simulink library "lib_AC_GFM"  (R2026a)
settings: Solver=VariableStepAuto
undefined symbols (not defined in the file): block_buses, block_idx, block_toM, buses_lf, fref, iC, invL, iR, iTf, op_GFM
libraries: simulink x4
(part 2 of 2)

== system lib_AC_GFM/GFM/VCC/dynamic_limiting/PIvd ==
  ref : Inport
  y : Inport  Port=2
  anti_windup : Inport  Port=3
  Gain : Gain  Gain=Bext
  Gain1 : Gain  Gain=1./Text
  Gain2 : Gain  Gain=Kext
  I : Integrator  InitialCondition=op_GFM.VCC_dynamic_limiting_PIvd_I
  Product : Product
  Scope : Scope
      settings: ActiveDisplayYMinimum=-5E-5  ActiveDisplayYMaximum=0.00079  DataLoggingVariableName=ScopeData5
  Scope1 : Scope
      settings: ActiveDisplayYMinimum=-0.29497  ActiveDisplayYMaximum=2.2504  DataLoggingVariableName=ScopeData7
  Sum : Sum  Inputs=++|
  Sum1 : Sum  Inputs=|+-
  Sum6 : Sum  Inputs=|+-
  Out1 : Outport
  wires:
  y/1 -> Sum1/2, Sum6/2
  ref/1 -> Gain/1, Sum6/1
  Gain/1 -> Sum1/1
  Sum/1 -> Gain2/1
  Sum1/1 -> Sum/1
  Sum6/1 -> Scope1/1, Gain1/1
  Product/1 -> I/1
  I/1 -> Scope/1, Sum/2
  Gain2/1 -> Out1/1
  Gain1/1 -> Product/1
  anti_windup/1 -> Product/2

== system lib_AC_GFM/GFM/VCC/dynamic_limiting/PIvq ==
  ref : Inport
  y : Inport  Port=2
  anti_windup : Inport  Port=3
  Gain : Gain  Gain=Bext
  Gain1 : Gain  Gain=1./Text
  Gain2 : Gain  Gain=Kext
  I : Integrator  InitialCondition=op_GFM.VCC_dynamic_limiting_PIvq_I
  Product : Product
  Sum : Sum  Inputs=++|
  Sum1 : Sum  Inputs=|+-
  Sum6 : Sum  Inputs=|+-
  Out1 : Outport
  wires:
  Gain2/1 -> Out1/1
  I/1 -> Sum/2
  Product/1 -> I/1
  Sum6/1 -> Gain1/1
  Sum1/1 -> Sum/1
  Sum/1 -> Gain2/1
  Gain/1 -> Sum1/1
  ref/1 -> Sum6/1, Gain/1
  y/1 -> Sum6/2, Sum1/2
  Gain1/1 -> Product/1
  anti_windup/1 -> Product/2

== system lib_AC_GFM/GFM/VCC/dynamic_limiting/RC ==
  note: 1) Add Subsystem or Model blocks as valid variant choices.
      | 2) You cannot connect blocks at this level. At simulation, connectivity is automatically
      | determined, based on the active variant and port name matching.
  i_d_in : Inport
  i_d_out : Inport  Port=2
  i_q_in : Inport  Port=3
  i_q_out : Inport  Port=4
  omega : Inport  Port=5
  dynamic : Subsystem  VariantControl=rc_mode == 1
  static : Subsystem  VariantControl=rc_mode == 2
  static omega : Subsystem  VariantControl=(default)
  vd : Outport
  vq : Outport  Port=2

== system lib_AC_GFM/GFM/VCC/dynamic_limiting/RL ==
  note: 1) Add Subsystem or Model blocks as valid variant choices.
      | 2) You cannot connect blocks at this level. At simulation, connectivity is automatically
      | determined, based on the active variant and port name matching.
  v_in_d : Inport
  v_out_d : Inport  Port=2
  v_in_q : Inport  Port=3
  v_out_q : Inport  Port=4
  omega : Inport  Port=5
  dynamic : Subsystem  VariantControl=rl_mode == 1
      settings: PortSchema="{\"entries\":[{\"content\":{\"sides\":[{\"content\":{\"connectorIds\":[\"In1\"]},\"type\":\"ConnectorPlacement.EquallySpacedRectSide\",\"uuid\":\"63966e24-f9e7-4b2d-b456-7f4ea5e3f230\"},{\"content\":{\"connectorIds\":[\"In2\",\"In3\",\"In4\",\"In5\",\"Out1\",\"Out2\"],\"side\":\"RIGHT\"},\"type\":\"ConnectorPlacement.EquallySpacedRectSide\",\"uuid\":\"ded6ef04-52fd-47df-8e49-cf16b827098d\"},{\"content\":{\"side\":\"TOP\"},\"type\":\"ConnectorPlacement.EquallySpacedRectSide\",\"uuid\":\"f940a985-fa23-4968-ad44-1d76d0e20c6a\"}]},\"type\":\"ConnectorPlacement.EquallySpacedConnector\",\"uuid\":\"20f61d3c-9af2-4982-98ea-af4910e61c9c\"}],\"packageUris\":[\"http://schema.mathworks.com/mf0/Connector/R2020b\"],\"version\":\"1.0\"}"
  static : Subsystem  VariantControl=rl_mode == 2
  static_omega : Subsystem  VariantControl=(default)
  id : Outport
  iq : Outport  Port=2

== system lib_AC_GFM/GFM/VCC/dynamic_limiting/VI ==
  id : Inport
  iq : Inport  Port=2
  Gain : Gain  Gain=L
  Gain1 : Gain  Gain=R
  Gain2 : Gain  Gain=L
  Gain3 : Gain  Gain=R
  LPF_omega : Subsystem
  LPF_omega1 : Subsystem
  Sum : Sum  Inputs=-+|
  Sum1 : Sum  Inputs=|--
  WOF_d : Subsystem  Variant=on
  WOF_q : Subsystem  Variant=on
  vd : Outport
  vq : Outport  Port=2
  wires:
  WOF_q/1(Out1) -> Gain/1, Gain3/1
  iq/1 -> WOF_q/1(In1)
  WOF_d/1(Out1) -> Gain1/1, Gain2/1
  id/1 -> WOF_d/1(In1)
  Sum1/1 -> LPF_omega1/1(in)
  Sum/1 -> LPF_omega/1(in)
  Gain3/1 -> Sum1/2
  Gain1/1 -> Sum/1
  Gain2/1 -> Sum1/1
  Gain/1 -> Sum/2
  LPF_omega/1(out) -> vd/1
  LPF_omega1/1(out) -> vq/1

== system lib_AC_GFM/GFM/VI/WOF_d/Active ==
  In1 : Inport
  Impl : Subsystem
  Out1 : Outport
  wires:
  Impl/1(Out1) -> Out1/1
  In1/1 -> Impl/1(In1)

== system lib_AC_GFM/GFM/VI/WOF_d/Bypass ==
  In1 : Inport
  Out1 : Outport
  wires:
  In1/1 -> Out1/1

== system lib_AC_GFM/GFM/VI/WOF_q/Active ==
  In1 : Inport
  Impl : Subsystem
  Out1 : Outport
  wires:
  Impl/1(Out1) -> Out1/1
  In1/1 -> Impl/1(In1)

== system lib_AC_GFM/GFM/VI/WOF_q/Bypass ==
  In1 : Inport
  Out1 : Outport
  wires:
  In1/1 -> Out1/1

== system lib_AC_GFM/GFM/PC/LPF_P/Active/Impl ==
  P : Inport
  Gain : Gain  Gain=iTf
  I : Integrator  InitialCondition=op_GFM.PC_LPF_P_Active_Impl_I
  Sum4 : Sum  Inputs=|+-
  P_f : Outport
  wires:
  I/1 -> Sum4/2, P_f/1
  P/1 -> Sum4/1
  Sum4/1 -> Gain/1
  Gain/1 -> I/1

== system lib_AC_GFM/GFM/PC/LPF_Q/Active/Impl ==
  Q : Inport
  Gain : Gain  Gain=iTf
  I : Integrator  InitialCondition=op_GFM.PC_LPF_Q_Active_Impl_I
  Sum4 : Sum  Inputs=|+-
  Q_f : Outport
  wires:
  Sum4/1 -> Gain/1
  I/1 -> Sum4/2, Q_f/1
  Q/1 -> Sum4/1
  Gain/1 -> I/1

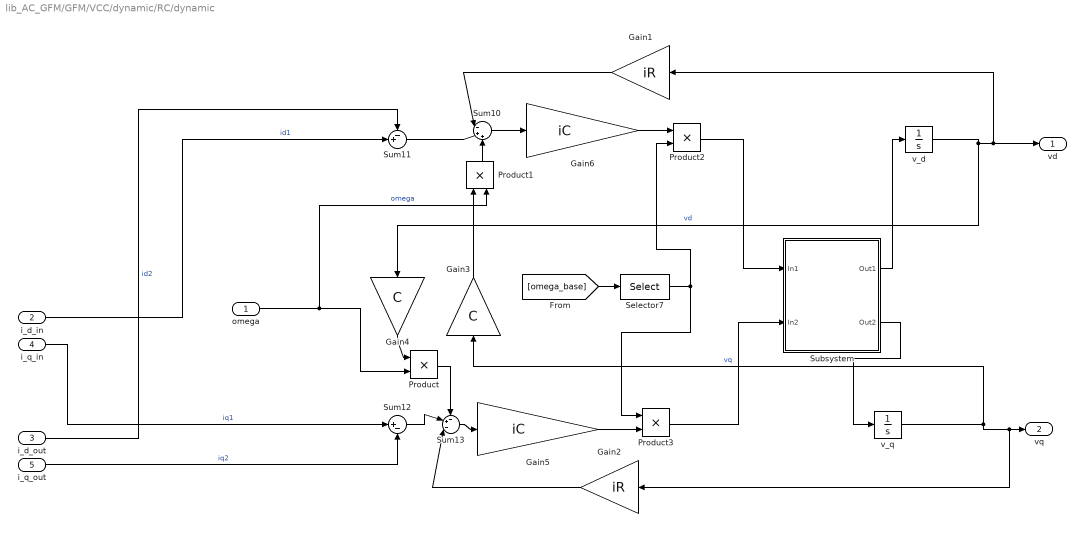
== system lib_AC_GFM/GFM/VCC/dynamic/RC/dynamic ==
  omega : Inport
  i_d_in : Inport  Port=2
  i_d_out : Inport  Port=3
  i_q_in : Inport  Port=4
  i_q_out : Inport  Port=5
  Gain1 : Gain  Gain=iR
  Gain2 : Gain  Gain=iR
  Gain3 : Gain  Gain=C
  Gain4 : Gain  Gain=C
  Gain5 : Gain  Gain=iC
  Gain6 : Gain  Gain=iC
  Product{,1..3} (4 alike) : Product
  Selector7 : Selector  InputPortWidth=length(fref.ref_units)  IndexOptions=Index vector (dialog)  Indices=block_fref  OutputSizes=1
  Subsystem : Subsystem
  Sum10 : Sum  Inputs=|-++
  Sum11 : Sum  Inputs=-+|
  Sum12 : Sum  Inputs=|+-
  Sum13 : Sum  Inputs=-+-|
  v_d : Integrator  InitialCondition=op_GFM.VCC_dynamic_RC_dynamic_v_d
  v_q : Integrator  InitialCondition=op_GFM.VCC_dynamic_RC_dynamic_v_q
  vd : Outport
  vq : Outport  Port=2
  wires:
  Sum10/1 -> Gain6/1
  Gain3/1 -> Product1/1
  v_q/1 -> vq/1, Gain2/1, Gain3/1  "vq"
  Product1/1 -> Sum10/3
  Gain4/1 -> Product/1
  Gain2/1 -> Sum13/3
  Product/1 -> Sum13/1
  Sum11/1 -> Sum10/2
  omega/1 -> Product/2, Product1/2  "omega"
  Sum13/1 -> Gain5/1
  Gain1/1 -> Sum10/1
  Sum12/1 -> Sum13/2
  v_d/1 -> Gain4/1, Gain1/1, vd/1  "vd"
  i_d_in/1 -> Sum11/2  "id1"
  i_d_out/1 -> Sum11/1  "id2"
  i_q_in/1 -> Sum12/1  "iq1"
  i_q_out/1 -> Sum12/2  "iq2"
  [omega_base] -> Selector7/1
  Gain6/1 -> Product2/1
  Product2/1 -> Subsystem/1(In1)
  Selector7/1 -> Product2/2, Product3/1
  Gain5/1 -> Product3/2
  Subsystem/1(Out1) -> v_d/1
  Product3/1 -> Subsystem/2(In2)
  Subsystem/2(Out2) -> v_q/1

== system lib_AC_GFM/GFM/VCC/dynamic/RC/static ==
  omega : Inport
  i_d_in : Inport  Port=2
  i_d_out : Inport  Port=3
  i_q_in : Inport  Port=4
  i_q_out : Inport  Port=5
  Constant : Constant  Value=iR.^2
  Constant1 : Constant
  Divide : Product  Inputs=*/
  Gain : Gain  Gain=C
  Gain1 : Gain  Gain=iR
  Gain2 : Gain  Gain=iR
  Product{,1..5} (6 alike) : Product
  Sum : Sum  Inputs=|++
  Sum1 : Sum  Inputs=|-+
  Sum2 : Sum  Inputs=|+-
  Sum3 : Sum  Inputs=|++
  Sum4 : Sum  Inputs=|-+
  vd : Outport
  vq : Outport  Port=2
  wires:
  Product5/1 -> Sum4/2
  Gain2/1 -> Product5/2
  Product4/1 -> Sum4/1
  Product2/1 -> Product3/1, Product4/2
  Product3/1 -> Sum3/2
  Product1/1 -> Sum3/1
  Divide/1 -> Product2/1, Gain1/1, Product5/1
  Gain1/1 -> Product1/2
  Sum2/1 -> Product3/2, Gain2/1  "iq"
  Sum1/1 -> Product4/1, Product1/1  "id"
  Constant1/1 -> Divide/1
  Product/1 -> Sum/2
  Gain/1 -> Product/1, Product/2, Product2/2
  Sum/1 -> Divide/2
  Constant/1 -> Sum/1
  Sum4/1 -> vq/1  "vq"
  Sum3/1 -> vd/1  "vd"
  omega/1 -> Gain/1  "omega"
  i_d_in/1 -> Sum1/2  "id1"
  i_q_in/1 -> Sum1/1  "id2"
  i_d_out/1 -> Sum2/1  "iq1"
  i_q_out/1 -> Sum2/2  "iq2"

== system lib_AC_GFM/GFM/VCC/dynamic/RC/static omega ==
  i_d_in : Inport
  i_d_out : Inport  Port=2
  i_q_in : Inport  Port=3
  i_q_out : Inport  Port=4
  Gain : Gain  Gain=1./(iR.^2+C.^2)
  Gain2 : Gain  Gain=1./(iR.^2+C.^2)
  Gain3 : Gain  Gain=iR
  Gain4 : Gain  Gain=C
  Gain5 : Gain  Gain=iR
  Gain6 : Gain  Gain=C
  Sum : Sum  Inputs=|++
  Sum1 : Sum  Inputs=|+-
  Sum2 : Sum  Inputs=|+-
  Sum4 : Sum  Inputs=|-+
  vd : Outport
  vq : Outport  Port=2
  wires:
  i_q_in/1 -> Sum2/1  "iq1"
  Sum1/1 -> Gain/1  "id"
  Sum2/1 -> Gain2/1  "iq"
  i_q_out/1 -> Sum2/2  "iq2"
  i_d_in/1 -> Sum1/1  "id"
  i_d_out/1 -> Sum1/2
  Gain/1 -> Gain4/1, Gain3/1
  Gain2/1 -> Gain6/1, Gain5/1
  Gain3/1 -> Sum/1
  Gain6/1 -> Sum/2
  Gain4/1 -> Sum4/1
  Gain5/1 -> Sum4/2
  Sum4/1 -> vq/1
  Sum/1 -> vd/1

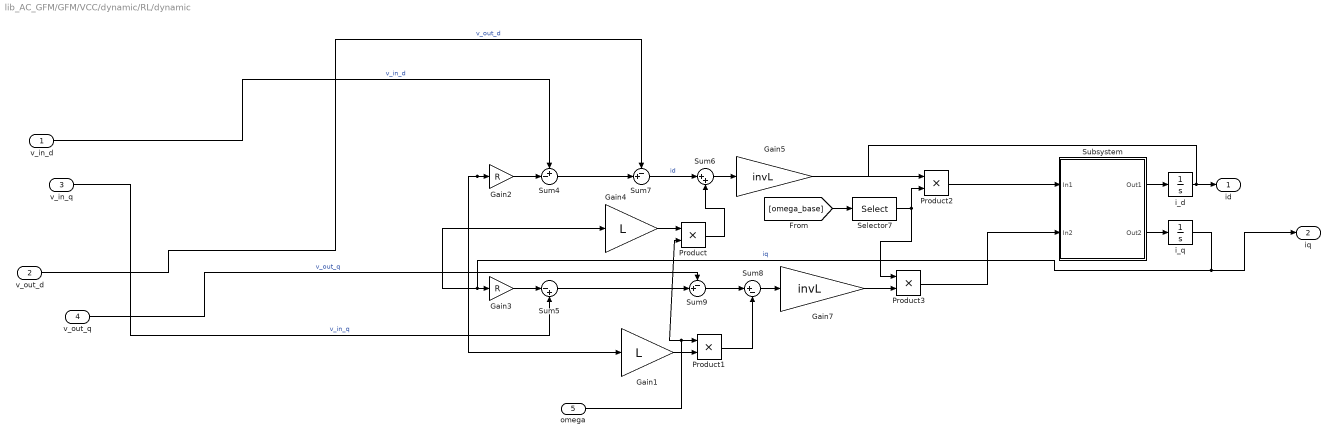
== system lib_AC_GFM/GFM/VCC/dynamic/RL/dynamic ==
  v_in_d : Inport
  v_out_d : Inport  Port=2
  v_in_q : Inport  Port=3
  v_out_q : Inport  Port=4
  omega : Inport  Port=5
  Gain1 : Gain  Gain=L
  Gain2 : Gain  Gain=R
  Gain3 : Gain  Gain=R
  Gain4 : Gain  Gain=L
  Gain5 : Gain  Gain=invL
  Gain7 : Gain  Gain=invL
  Product{,1..3} (4 alike) : Product
  Selector7 : Selector  InputPortWidth=length(fref.ref_units)  IndexOptions=Index vector (dialog)  Indices=block_fref  OutputSizes=1
  Subsystem : Subsystem
  Sum4 : Sum  Inputs=+-|
  Sum5 : Sum  Inputs=|-+
  Sum6 : Sum  Inputs=|++
  Sum7 : Sum  Inputs=-+|
  Sum8 : Sum  Inputs=|+-
  Sum9 : Sum  Inputs=-+|
  i_d : Integrator  InitialCondition=op_GFM.VCC_dynamic_RL_dynamic_i_d
  i_q : Integrator  InitialCondition=op_GFM.VCC_dynamic_RL_dynamic_i_q
  id : Outport
  iq : Outport  Port=2
  wires:
  v_out_q/1 -> Sum9/1  "v_out_q"
  v_out_d/1 -> Sum7/1  "v_out_d"
  Sum9/1 -> Sum8/1
  Gain1/1 -> Product1/2
  i_q/1 -> Gain4/1, Gain3/1, iq/1  "iq"
  Gain7/1 -> Product3/2
  Sum5/1 -> Sum9/2
  Gain3/1 -> Sum5/1
  Sum7/1 -> Sum6/1
  Gain4/1 -> Product/1
  Product1/1 -> Sum8/2
  Sum4/1 -> Sum7/2
  Sum8/1 -> Gain7/1
  Product/1 -> Sum6/2
  Sum6/1 -> Gain5/1
  i_d/1 -> id/1, Gain1/1, Gain2/1  "id"
  Gain2/1 -> Sum4/2
  v_in_d/1 -> Sum4/1  "v_in_d"
  v_in_q/1 -> Sum5/2  "v_in_q"
  omega/1 -> Product/2, Product1/1
  Gain5/1 -> Product2/1
  Product2/1 -> Subsystem/1(In1)
  Selector7/1 -> Product2/2, Product3/1
  [omega_base] -> Selector7/1
  Product3/1 -> Subsystem/2(In2)
  Subsystem/1(Out1) -> i_d/1
  Subsystem/2(Out2) -> i_q/1

== system lib_AC_GFM/GFM/VCC/dynamic/RL/static ==
  v_in_d : Inport
  v_out_d : Inport  Port=2
  v_in_q : Inport  Port=3
  v_out_q : Inport  Port=4
  omega : Inport  Port=5
  Constant : Constant  Value=R.^2
  Constant1 : Constant
  Divide : Product  Inputs=*/
  Gain : Gain  Gain=L
  Gain1 : Gain  Gain=R
  Gain2 : Gain  Gain=R
  Product{,1..5} (6 alike) : Product
  Sum : Sum  Inputs=|++
  Sum1 : Sum  Inputs=|+-
  Sum2 : Sum  Inputs=|+-
  Sum3 : Sum  Inputs=|++
  Sum4 : Sum  Inputs=|-+
  id : Outport
  iq : Outport  Port=2
  wires:
  omega/1 -> Gain/1  "omega"
  v_in_d/1 -> Sum1/1  "v_in_d"
  v_out_q/1 -> Sum2/2  "v_out_q"
  Sum4/1 -> iq/1  "iq"
  Sum3/1 -> id/1  "id"
  Gain1/1 -> Product1/2
  Product2/1 -> Product4/2, Product3/1
  Product4/1 -> Sum4/1
  Divide/1 -> Gain2/1, Gain1/1, Product2/1
  Sum1/1 -> Product1/1, Product4/1  "vd"
  Product3/1 -> Sum3/2
  Constant1/1 -> Divide/1
  Gain/1 -> Product/2, Product/1, Product2/2
  Sum2/1 -> Product5/1, Product3/2  "vq"
  Constant/1 -> Sum/1
  Product5/1 -> Sum4/2
  Product1/1 -> Sum3/1
  Product/1 -> Sum/2
  Gain2/1 -> Product5/2
  Sum/1 -> Divide/2
  v_out_d/1 -> Sum1/2  "v_out_d"
  v_in_q/1 -> Sum2/1  "v_in_q"

== system lib_AC_GFM/GFM/VCC/dynamic/RL/static_omega ==
  v_in_d : Inport
  v_out_d : Inport  Port=2
  v_in_q : Inport  Port=3
  v_out_q : Inport  Port=4
  Gain : Gain  Gain=1./(R.^2+L.^2)
  Gain2 : Gain  Gain=1./(R.^2+L.^2)
  Gain3 : Gain  Gain=R
  Gain4 : Gain  Gain=L
  Gain5 : Gain  Gain=L
  Gain6 : Gain  Gain=R
  Sum : Sum  Inputs=|++
  Sum1 : Sum  Inputs=|+-
  Sum2 : Sum  Inputs=|+-
  Sum3 : Sum  Inputs=|-+
  id : Outport
  iq : Outport  Port=2
  wires:
  v_in_q/1 -> Sum2/1  "v_in_q"
  v_in_d/1 -> Sum1/1  "v_in_d"
  v_out_q/1 -> Sum2/2  "v_out_q"
  v_out_d/1 -> Sum1/2  "v_out_d"
  Sum1/1 -> Gain/1  "vd"
  Sum2/1 -> Gain2/1  "vq"
  Gain/1 -> Gain5/1, Gain3/1
  Gain3/1 -> Sum/1
  Gain4/1 -> Sum/2
  Gain2/1 -> Gain6/1, Gain4/1
  Sum/1 -> id/1
  Gain5/1 -> Sum3/1
  Sum3/1 -> iq/1
  Gain6/1 -> Sum3/2

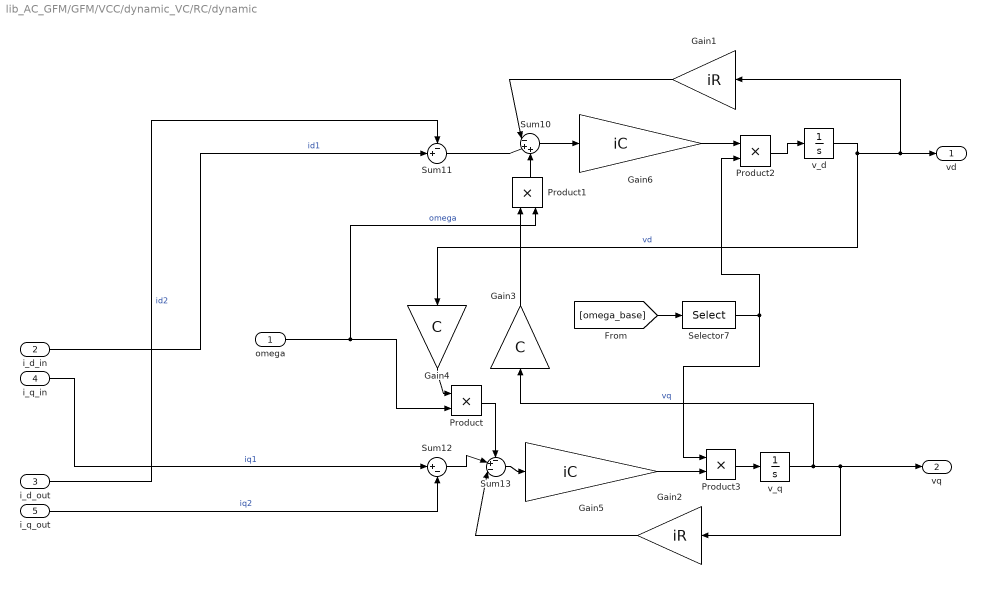
== system lib_AC_GFM/GFM/VCC/dynamic_VC/RC/dynamic ==
  omega : Inport
  i_d_in : Inport  Port=2
  i_d_out : Inport  Port=3
  i_q_in : Inport  Port=4
  i_q_out : Inport  Port=5
  Gain1 : Gain  Gain=iR
  Gain2 : Gain  Gain=iR
  Gain3 : Gain  Gain=C
  Gain4 : Gain  Gain=C
  Gain5 : Gain  Gain=iC
  Gain6 : Gain  Gain=iC
  Product{,1..3} (4 alike) : Product
  Selector7 : Selector  InputPortWidth=length(fref.ref_units)  IndexOptions=Index vector (dialog)  Indices=block_fref  OutputSizes=1
  Sum10 : Sum  Inputs=|-++
  Sum11 : Sum  Inputs=-+|
  Sum12 : Sum  Inputs=|+-
  Sum13 : Sum  Inputs=-+-|
  v_d : Integrator  InitialCondition=op_GFM.VCC_dynamic_VC_RC_dynamic_v_d
  v_q : Integrator  InitialCondition=op_GFM.VCC_dynamic_VC_RC_dynamic_v_q
  vd : Outport
  vq : Outport  Port=2
  wires:
  Sum10/1 -> Gain6/1
  Gain3/1 -> Product1/1
  v_q/1 -> vq/1, Gain2/1, Gain3/1  "vq"
  Product1/1 -> Sum10/3
  Gain4/1 -> Product/1
  Gain2/1 -> Sum13/3
  Product/1 -> Sum13/1
  Sum11/1 -> Sum10/2
  omega/1 -> Product/2, Product1/2  "omega"
  Sum13/1 -> Gain5/1
  Gain1/1 -> Sum10/1
  Sum12/1 -> Sum13/2
  v_d/1 -> Gain4/1, vd/1, Gain1/1  "vd"
  i_d_in/1 -> Sum11/2  "id1"
  i_d_out/1 -> Sum11/1  "id2"
  i_q_in/1 -> Sum12/1  "iq1"
  i_q_out/1 -> Sum12/2  "iq2"
  [omega_base] -> Selector7/1
  Gain6/1 -> Product2/1
  Product2/1 -> v_d/1
  Selector7/1 -> Product2/2, Product3/1
  Product3/1 -> v_q/1
  Gain5/1 -> Product3/2

== system lib_AC_GFM/GFM/VCC/dynamic_VC/RC/static ==
  omega : Inport
  i_d_in : Inport  Port=2
  i_d_out : Inport  Port=3
  i_q_in : Inport  Port=4
  i_q_out : Inport  Port=5
  Constant : Constant  Value=iR.^2
  Constant1 : Constant
  Divide : Product  Inputs=*/
  Gain : Gain  Gain=C
  Gain1 : Gain  Gain=iR
  Gain2 : Gain  Gain=iR
  Product{,1..5} (6 alike) : Product
  Sum : Sum  Inputs=|++
  Sum1 : Sum  Inputs=|-+
  Sum2 : Sum  Inputs=|+-
  Sum3 : Sum  Inputs=|++
  Sum4 : Sum  Inputs=|-+
  vd : Outport
  vq : Outport  Port=2
  wires:
  Product5/1 -> Sum4/2
  Gain2/1 -> Product5/2
  Product4/1 -> Sum4/1
  Product2/1 -> Product3/1, Product4/2
  Product3/1 -> Sum3/2
  Product1/1 -> Sum3/1
  Divide/1 -> Product2/1, Gain1/1, Product5/1
  Gain1/1 -> Product1/2
  Sum2/1 -> Product3/2, Gain2/1  "iq"
  Sum1/1 -> Product4/1, Product1/1  "id"
  Constant1/1 -> Divide/1
  Product/1 -> Sum/2
  Gain/1 -> Product/1, Product/2, Product2/2
  Sum/1 -> Divide/2
  Constant/1 -> Sum/1
  Sum4/1 -> vq/1  "vq"
  Sum3/1 -> vd/1  "vd"
  omega/1 -> Gain/1  "omega"
  i_d_in/1 -> Sum1/2  "id1"
  i_q_in/1 -> Sum1/1  "id2"
  i_d_out/1 -> Sum2/1  "iq1"
  i_q_out/1 -> Sum2/2  "iq2"

== system lib_AC_GFM/GFM/VCC/dynamic_VC/RC/static omega ==
  i_d_in : Inport
  i_d_out : Inport  Port=2
  i_q_in : Inport  Port=3
  i_q_out : Inport  Port=4
  Gain : Gain  Gain=1./(iR.^2+C.^2)
  Gain2 : Gain  Gain=1./(iR.^2+C.^2)
  Gain3 : Gain  Gain=iR
  Gain4 : Gain  Gain=C
  Gain5 : Gain  Gain=iR
  Gain6 : Gain  Gain=C
  Sum : Sum  Inputs=|++
  Sum1 : Sum  Inputs=|+-
  Sum2 : Sum  Inputs=|+-
  Sum4 : Sum  Inputs=|-+
  vd : Outport
  vq : Outport  Port=2
  wires:
  i_q_in/1 -> Sum2/1  "iq1"
  Sum1/1 -> Gain/1  "id"
  Sum2/1 -> Gain2/1  "iq"
  i_q_out/1 -> Sum2/2  "iq2"
  i_d_in/1 -> Sum1/1  "id"
  i_d_out/1 -> Sum1/2
  Gain/1 -> Gain4/1, Gain3/1
  Gain2/1 -> Gain6/1, Gain5/1
  Gain3/1 -> Sum/1
  Gain6/1 -> Sum/2
  Gain4/1 -> Sum4/1
  Gain5/1 -> Sum4/2
  Sum4/1 -> vq/1
  Sum/1 -> vd/1

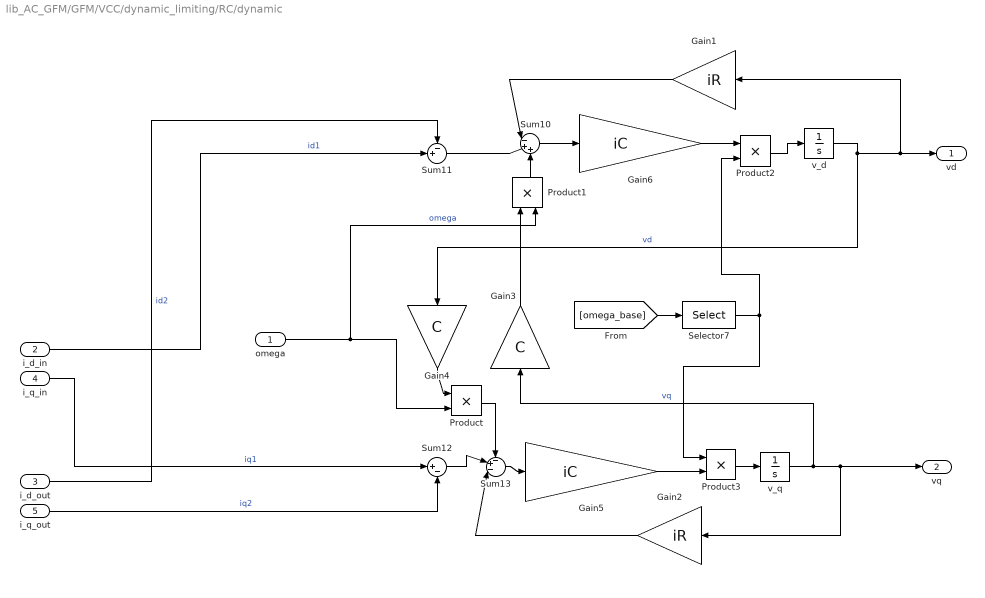
== system lib_AC_GFM/GFM/VCC/dynamic_limiting/RC/dynamic ==
  omega : Inport
  i_d_in : Inport  Port=2
  i_d_out : Inport  Port=3
  i_q_in : Inport  Port=4
  i_q_out : Inport  Port=5
  Gain1 : Gain  Gain=iR
  Gain2 : Gain  Gain=iR
  Gain3 : Gain  Gain=C
  Gain4 : Gain  Gain=C
  Gain5 : Gain  Gain=iC
  Gain6 : Gain  Gain=iC
  Product{,1..3} (4 alike) : Product
  Selector7 : Selector  InputPortWidth=length(fref.ref_units)  IndexOptions=Index vector (dialog)  Indices=block_fref  OutputSizes=1
  Sum10 : Sum  Inputs=|-++
  Sum11 : Sum  Inputs=-+|
  Sum12 : Sum  Inputs=|+-
  Sum13 : Sum  Inputs=-+-|
  v_d : Integrator  InitialCondition=op_GFM.VCC_dynamic_limiting_RC_dynamic_v_d
  v_q : Integrator  InitialCondition=op_GFM.VCC_dynamic_limiting_RC_dynamic_v_q
  vd : Outport
  vq : Outport  Port=2
  wires:
  Sum10/1 -> Gain6/1
  Gain3/1 -> Product1/1
  v_q/1 -> vq/1, Gain2/1, Gain3/1  "vq"
  Product1/1 -> Sum10/3
  Gain4/1 -> Product/1
  Gain2/1 -> Sum13/3
  Product/1 -> Sum13/1
  Sum11/1 -> Sum10/2
  omega/1 -> Product/2, Product1/2  "omega"
  Sum13/1 -> Gain5/1
  Gain1/1 -> Sum10/1
  Sum12/1 -> Sum13/2
  v_d/1 -> Gain4/1, vd/1, Gain1/1  "vd"
  i_d_in/1 -> Sum11/2  "id1"
  i_d_out/1 -> Sum11/1  "id2"
  i_q_in/1 -> Sum12/1  "iq1"
  i_q_out/1 -> Sum12/2  "iq2"
  [omega_base] -> Selector7/1
  Gain6/1 -> Product2/1
  Product2/1 -> v_d/1
  Selector7/1 -> Product2/2, Product3/1
  Product3/1 -> v_q/1
  Gain5/1 -> Product3/2

== system lib_AC_GFM/GFM/VCC/dynamic_limiting/RC/static ==
  omega : Inport
  i_d_in : Inport  Port=2
  i_d_out : Inport  Port=3
  i_q_in : Inport  Port=4
  i_q_out : Inport  Port=5
  Constant : Constant  Value=iR.^2
  Constant1 : Constant
  Divide : Product  Inputs=*/
  Gain : Gain  Gain=C
  Gain1 : Gain  Gain=iR
  Gain2 : Gain  Gain=iR
  Product{,1..5} (6 alike) : Product
  Sum : Sum  Inputs=|++
  Sum1 : Sum  Inputs=|-+
  Sum2 : Sum  Inputs=|+-
  Sum3 : Sum  Inputs=|++
  Sum4 : Sum  Inputs=|-+
  vd : Outport
  vq : Outport  Port=2
  wires:
  Product5/1 -> Sum4/2
  Gain2/1 -> Product5/2
  Product4/1 -> Sum4/1
  Product2/1 -> Product3/1, Product4/2
  Product3/1 -> Sum3/2
  Product1/1 -> Sum3/1
  Divide/1 -> Product2/1, Gain1/1, Product5/1
  Gain1/1 -> Product1/2
  Sum2/1 -> Product3/2, Gain2/1  "iq"
  Sum1/1 -> Product4/1, Product1/1  "id"
  Constant1/1 -> Divide/1
  Product/1 -> Sum/2
  Gain/1 -> Product/1, Product/2, Product2/2
  Sum/1 -> Divide/2
  Constant/1 -> Sum/1
  Sum4/1 -> vq/1  "vq"
  Sum3/1 -> vd/1  "vd"
  omega/1 -> Gain/1  "omega"
  i_d_in/1 -> Sum1/2  "id1"
  i_q_in/1 -> Sum1/1  "id2"
  i_d_out/1 -> Sum2/1  "iq1"
  i_q_out/1 -> Sum2/2  "iq2"

== system lib_AC_GFM/GFM/VCC/dynamic_limiting/RC/static omega ==
  i_d_in : Inport
  i_d_out : Inport  Port=2
  i_q_in : Inport  Port=3
  i_q_out : Inport  Port=4
  Gain : Gain  Gain=1./(iR.^2+C.^2)
  Gain2 : Gain  Gain=1./(iR.^2+C.^2)
  Gain3 : Gain  Gain=iR
  Gain4 : Gain  Gain=C
  Gain5 : Gain  Gain=iR
  Gain6 : Gain  Gain=C
  Sum : Sum  Inputs=|++
  Sum1 : Sum  Inputs=|+-
  Sum2 : Sum  Inputs=|+-
  Sum4 : Sum  Inputs=|-+
  vd : Outport
  vq : Outport  Port=2
  wires:
  i_q_in/1 -> Sum2/1  "iq1"
  Sum1/1 -> Gain/1  "id"
  Sum2/1 -> Gain2/1  "iq"
  i_q_out/1 -> Sum2/2  "iq2"
  i_d_in/1 -> Sum1/1  "id"
  i_d_out/1 -> Sum1/2
  Gain/1 -> Gain4/1, Gain3/1
  Gain2/1 -> Gain6/1, Gain5/1
  Gain3/1 -> Sum/1
  Gain6/1 -> Sum/2
  Gain4/1 -> Sum4/1
  Gain5/1 -> Sum4/2
  Sum4/1 -> vq/1
  Sum/1 -> vd/1

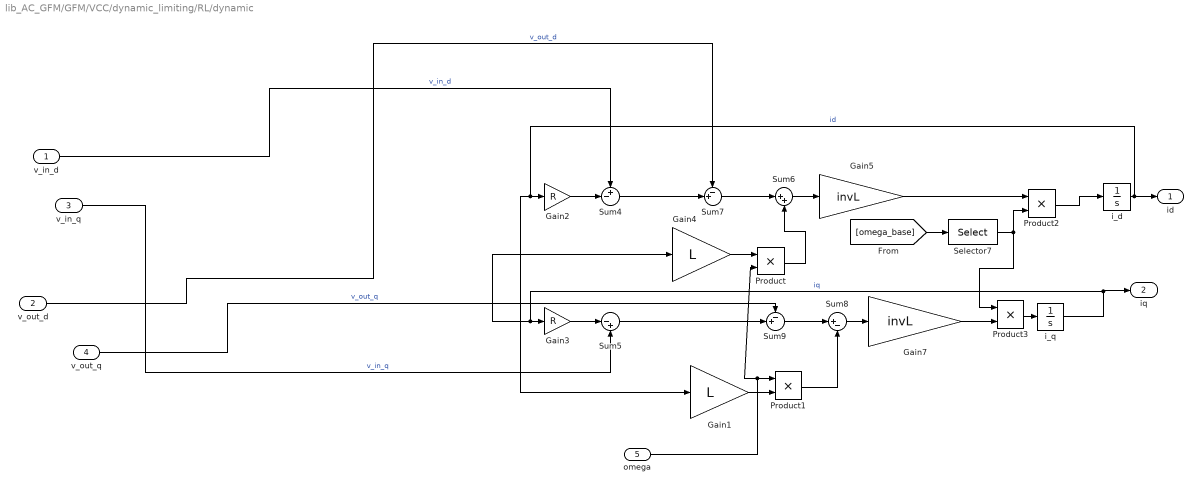
== system lib_AC_GFM/GFM/VCC/dynamic_limiting/RL/dynamic ==
  v_in_d : Inport
  v_out_d : Inport  Port=2
  v_in_q : Inport  Port=3
  v_out_q : Inport  Port=4
  omega : Inport  Port=5
  Gain1 : Gain  Gain=L
  Gain2 : Gain  Gain=R
  Gain3 : Gain  Gain=R
  Gain4 : Gain  Gain=L
  Gain5 : Gain  Gain=invL
  Gain7 : Gain  Gain=invL
  Product{,1..3} (4 alike) : Product
  Selector7 : Selector  InputPortWidth=length(fref.ref_units)  IndexOptions=Index vector (dialog)  Indices=block_fref  OutputSizes=1
  Sum4 : Sum  Inputs=+-|
  Sum5 : Sum  Inputs=|-+
  Sum6 : Sum  Inputs=|++
  Sum7 : Sum  Inputs=-+|
  Sum8 : Sum  Inputs=|+-
  Sum9 : Sum  Inputs=-+|
  i_d : Integrator  InitialCondition=op_GFM.VCC_dynamic_limiting_RL_dynamic_i_d
  i_q : Integrator  InitialCondition=op_GFM.VCC_dynamic_limiting_RL_dynamic_i_q
  id : Outport
  iq : Outport  Port=2
  wires:
  v_out_q/1 -> Sum9/1  "v_out_q"
  v_out_d/1 -> Sum7/1  "v_out_d"
  Sum9/1 -> Sum8/1
  Gain1/1 -> Product1/2
  i_q/1 -> iq/1, Gain4/1, Gain3/1  "iq"
  Gain7/1 -> Product3/2
  Sum5/1 -> Sum9/2
  Gain3/1 -> Sum5/1
  Sum7/1 -> Sum6/1
  Gain4/1 -> Product/1
  Product1/1 -> Sum8/2
  Sum4/1 -> Sum7/2
  Sum8/1 -> Gain7/1
  Product/1 -> Sum6/2
  Sum6/1 -> Gain5/1
  i_d/1 -> id/1, Gain1/1, Gain2/1  "id"
  Gain2/1 -> Sum4/2
  v_in_d/1 -> Sum4/1  "v_in_d"
  v_in_q/1 -> Sum5/2  "v_in_q"
  omega/1 -> Product/2, Product1/1
  Gain5/1 -> Product2/1
  Product2/1 -> i_d/1
  Selector7/1 -> Product2/2, Product3/1
  [omega_base] -> Selector7/1
  Product3/1 -> i_q/1

== system lib_AC_GFM/GFM/VCC/dynamic_limiting/RL/static ==
  v_in_d : Inport
  v_out_d : Inport  Port=2
  v_in_q : Inport  Port=3
  v_out_q : Inport  Port=4
  omega : Inport  Port=5
  Constant : Constant  Value=R.^2
  Constant1 : Constant
  Divide : Product  Inputs=*/
  Gain : Gain  Gain=L
  Gain1 : Gain  Gain=R
  Gain2 : Gain  Gain=R
  Product{,1..5} (6 alike) : Product
  Sum : Sum  Inputs=|++
  Sum1 : Sum  Inputs=|+-
  Sum2 : Sum  Inputs=|+-
  Sum3 : Sum  Inputs=|++
  Sum4 : Sum  Inputs=|-+
  id : Outport
  iq : Outport  Port=2
  wires:
  omega/1 -> Gain/1  "omega"
  v_in_d/1 -> Sum1/1  "v_in_d"
  v_out_q/1 -> Sum2/2  "v_out_q"
  Sum4/1 -> iq/1  "iq"
  Sum3/1 -> id/1  "id"
  Gain1/1 -> Product1/2
  Product2/1 -> Product4/2, Product3/1
  Product4/1 -> Sum4/1
  Divide/1 -> Gain2/1, Gain1/1, Product2/1
  Sum1/1 -> Product1/1, Product4/1  "vd"
  Product3/1 -> Sum3/2
  Constant1/1 -> Divide/1
  Gain/1 -> Product/2, Product/1, Product2/2
  Sum2/1 -> Product5/1, Product3/2  "vq"
  Constant/1 -> Sum/1
  Product5/1 -> Sum4/2
  Product1/1 -> Sum3/1
  Product/1 -> Sum/2
  Gain2/1 -> Product5/2
  Sum/1 -> Divide/2
  v_out_d/1 -> Sum1/2  "v_out_d"
  v_in_q/1 -> Sum2/1  "v_in_q"

== system lib_AC_GFM/GFM/VCC/dynamic_limiting/RL/static_omega ==
  v_in_d : Inport
  v_out_d : Inport  Port=2
  v_in_q : Inport  Port=3
  v_out_q : Inport  Port=4
  Gain : Gain  Gain=1./(R.^2+L.^2)
  Gain2 : Gain  Gain=1./(R.^2+L.^2)
  Gain3 : Gain  Gain=R
  Gain4 : Gain  Gain=L
  Gain5 : Gain  Gain=L
  Gain6 : Gain  Gain=R
  Sum : Sum  Inputs=|++
  Sum1 : Sum  Inputs=|+-
  Sum2 : Sum  Inputs=|+-
  Sum3 : Sum  Inputs=|-+
  id : Outport
  iq : Outport  Port=2
  wires:
  v_in_q/1 -> Sum2/1  "v_in_q"
  v_in_d/1 -> Sum1/1  "v_in_d"
  v_out_q/1 -> Sum2/2  "v_out_q"
  v_out_d/1 -> Sum1/2  "v_out_d"
  Sum1/1 -> Gain/1  "vd"
  Sum2/1 -> Gain2/1  "vq"
  Gain/1 -> Gain5/1, Gain3/1
  Gain3/1 -> Sum/1
  Gain4/1 -> Sum/2
  Gain2/1 -> Gain6/1, Gain4/1
  Sum/1 -> id/1
  Gain5/1 -> Sum3/1
  Sum3/1 -> iq/1
  Gain6/1 -> Sum3/2

== system lib_AC_GFM/GFM/VCC/dynamic_limiting/VI/LPF_omega ==
  in : Inport
  Gain : Gain  Gain=10
  I : Integrator  InitialCondition=op_GFM.VCC_dynamic_limiting_VI_LPF_omega_I
  Sum4 : Sum  Inputs=|+-
  out : Outport
  wires:
  Gain/1 -> I/1
  Sum4/1 -> Gain/1
  in/1 -> Sum4/1
  I/1 -> Sum4/2, out/1

== system lib_AC_GFM/GFM/VCC/dynamic_limiting/VI/LPF_omega1 ==
  in : Inport
  Gain : Gain  Gain=10
  I : Integrator  InitialCondition=op_GFM.VCC_dynamic_limiting_VI_LPF_omega1_I
  Sum4 : Sum  Inputs=|+-
  out : Outport
  wires:
  I/1 -> out/1, Sum4/2
  in/1 -> Sum4/1
  Sum4/1 -> Gain/1
  Gain/1 -> I/1

== system lib_AC_GFM/GFM/VCC/dynamic_limiting/VI/WOF_d ==
  note: 1) Add Subsystem or Model blocks as valid variant choices.
      | 2) You cannot connect blocks at this level. At simulation, connectivity is automatically
      | determined, based on the active variant and port name matching.
  In1 : Inport
  Active : Subsystem  VariantControl=use_Tf == 1
  Bypass : Subsystem  VariantControl=(default)
  Out1 : Outport

== system lib_AC_GFM/GFM/VCC/dynamic_limiting/VI/WOF_q ==
  note: 1) Add Subsystem or Model blocks as valid variant choices.
      | 2) You cannot connect blocks at this level. At simulation, connectivity is automatically
      | determined, based on the active variant and port name matching.
  In1 : Inport
  Active : Subsystem  VariantControl=use_Tf == 1
  Bypass : Subsystem  VariantControl=(default)
  Out1 : Outport

== system lib_AC_GFM/GFM/VI/WOF_d/Active/Impl ==
  In1 : Inport
  Gain : Gain  Gain=iTf
  I : Integrator  InitialConditionSource=external  InitialCondition=op_GFM.VI_WOF_d_Active_Impl_I
  Sum : Sum  Inputs=+-|
  Sum4 : Sum  Inputs=|+-
  Out1 : Outport
  wires:
  Gain/1 -> I/1
  Sum4/1 -> Gain/1
  In1/1 -> I/2, Sum/1, Sum4/1
  I/1 -> Sum/2, Sum4/2
  Sum/1 -> Out1/1

== system lib_AC_GFM/GFM/VI/WOF_q/Active/Impl ==
  In1 : Inport
  Gain : Gain  Gain=iTf
  I : Integrator  InitialConditionSource=external  InitialCondition=op_GFM.VI_WOF_q_Active_Impl_I
  Sum : Sum  Inputs=+-|
  Sum4 : Sum  Inputs=|+-
  Out1 : Outport
  wires:
  Gain/1 -> I/1
  Sum4/1 -> Gain/1
  In1/1 -> I/2, Sum/1, Sum4/1
  I/1 -> Sum/2, Sum4/2
  Sum/1 -> Out1/1

== system lib_AC_GFM/GFM/VCC/dynamic/RC/dynamic/Subsystem ==
  In1 : Inport
  In2 : Inport  Port=2
  Constant : Constant  Value=Text==Inf  VectorParams1D=off
  Switch : Switch  Criteria=u2 > Threshold  SaturateOnIntegerOverflow=off  InputSameDT=off
  Switch1 : Switch  Criteria=u2 > Threshold  SaturateOnIntegerOverflow=off  InputSameDT=off
  Zero : Constant  Value=0  OutDataTypeStr=Inherit: Inherit via back propagation
  Out1 : Outport
  Out2 : Outport  Port=2
  wires:
  Switch1/1 -> Out2/1
  Constant/1 -> Switch1/2, Switch/2
  Zero/1 -> Switch1/1, Switch/1
  In1/1 -> Switch/3
  Switch/1 -> Out1/1
  In2/1 -> Switch1/3

== system lib_AC_GFM/GFM/VCC/dynamic/RL/dynamic/Subsystem ==
  In1 : Inport
  In2 : Inport  Port=2
  Constant : Constant  Value=Tint==Inf  VectorParams1D=off
  Switch : Switch  Criteria=u2 > Threshold  SaturateOnIntegerOverflow=off  InputSameDT=off
  Switch1 : Switch  Criteria=u2 > Threshold  SaturateOnIntegerOverflow=off  InputSameDT=off
  Zero : Constant  Value=0  OutDataTypeStr=Inherit: Inherit via back propagation
  Out1 : Outport
  Out2 : Outport  Port=2
  wires:
  Switch1/1 -> Out2/1
  Constant/1 -> Switch1/2, Switch/2
  Zero/1 -> Switch1/1, Switch/1
  In1/1 -> Switch/3
  Switch/1 -> Out1/1
  In2/1 -> Switch1/3

== system lib_AC_GFM/GFM/VCC/dynamic_limiting/VI/WOF_d/Active ==
  In1 : Inport
  Impl : Subsystem
  Out1 : Outport
  wires:
  Impl/1(Out1) -> Out1/1
  In1/1 -> Impl/1(In1)

== system lib_AC_GFM/GFM/VCC/dynamic_limiting/VI/WOF_d/Bypass ==
  In1 : Inport
  Out1 : Outport
  wires:
  In1/1 -> Out1/1

== system lib_AC_GFM/GFM/VCC/dynamic_limiting/VI/WOF_q/Active ==
  In1 : Inport
  Impl : Subsystem
  Out1 : Outport
  wires:
  Impl/1(Out1) -> Out1/1
  In1/1 -> Impl/1(In1)

== system lib_AC_GFM/GFM/VCC/dynamic_limiting/VI/WOF_q/Bypass ==
  In1 : Inport
  Out1 : Outport
  wires:
  In1/1 -> Out1/1

== system lib_AC_GFM/GFM/VCC/dynamic_limiting/VI/WOF_d/Active/Impl ==
  In1 : Inport
  Gain : Gain  Gain=iTf
  I : Integrator  InitialConditionSource=external  InitialCondition=op_GFM.VCC_dynamic_limiting_VI_WOF_d_Active_Impl_I
  Sum : Sum  Inputs=+-|
  Sum4 : Sum  Inputs=|+-
  Out1 : Outport
  wires:
  Gain/1 -> I/1
  Sum4/1 -> Gain/1
  In1/1 -> I/2, Sum/1, Sum4/1
  I/1 -> Sum/2, Sum4/2
  Sum/1 -> Out1/1

== system lib_AC_GFM/GFM/VCC/dynamic_limiting/VI/WOF_q/Active/Impl ==
  In1 : Inport
  Gain : Gain  Gain=iTf
  I : Integrator  InitialConditionSource=external  InitialCondition=op_GFM.VCC_dynamic_limiting_VI_WOF_q_Active_Impl_I
  Sum : Sum  Inputs=+-|
  Sum4 : Sum  Inputs=|+-
  Out1 : Outport
  wires:
  Gain/1 -> I/1
  Sum4/1 -> Gain/1
  In1/1 -> I/2, Sum/1, Sum4/1
  I/1 -> Sum/2, Sum4/2
  Sum/1 -> Out1/1
